simulink subsystem "est_observer"  (R2023a)
settings: Solver=VariableStepAuto  StartTime=0.0  StopTime=10.0  RelTol=1e-3
undefined symbols (not defined in the file or in its folder): ctrlP
libraries: simulink x1
settings Model: Creator=ahmad  LastModifiedBy=ahmad
settings ModelReferenceCC: UpdateModelReferenceTargets=IfOutOfDate
settings RTWCC: GPUComputeCapability=5.0
settings ConfigComp: CovBoundaryAbsTol=1.0e-5

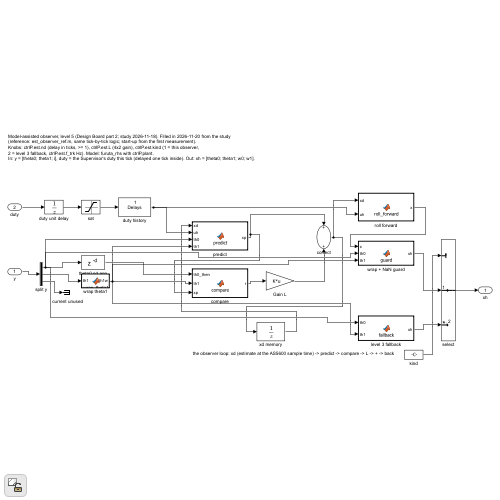
[thumbnail: Simulink's stored preview of the top-level diagram]
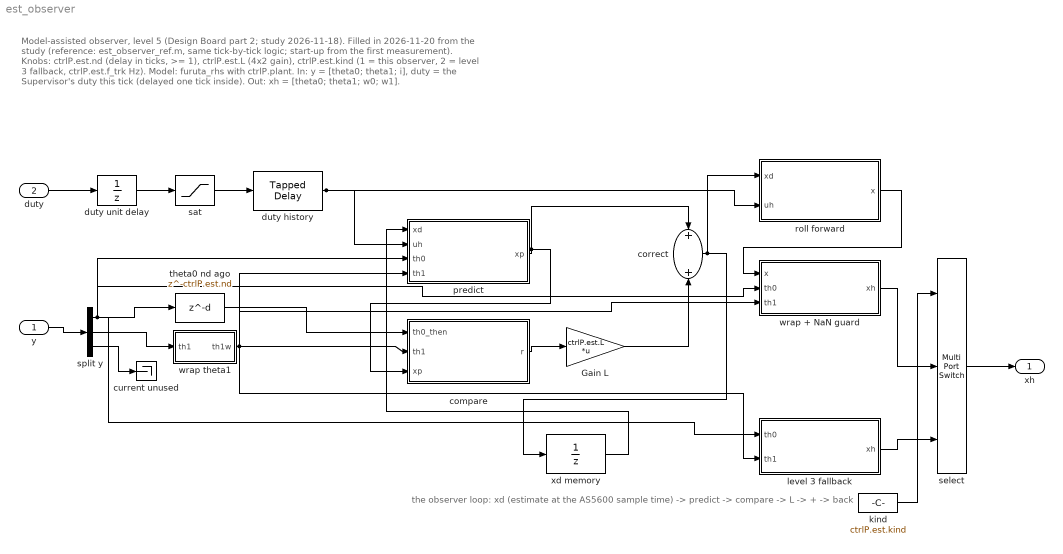
== system est_observer ==
  note: Model-assisted observer, level 5 (Design Board part 2; study 2026-11-18). Filled in 2026-11-20 from the study
      | (reference: est_observer_ref.m, same tick-by-tick logic; start-up from the first measurement).
      | Knobs: ctrlP.est.nd (delay in ticks, >= 1), ctrlP.est.L (4x2 gain), ctrlP.est.kind (1 = this observer,
      | 2 = level 3 fallback, ctrlP.est.f_trk Hz). Model: furuta_rhs with ctrlP.plant.
      | In: y = [theta0; theta1; i], duty = the Supervisor's duty this tick (delayed one tick inside). Out: xh = [theta0; theta1; w0; w1].
  note: the observer loop: xd (estimate at the AS5600 sample time) -> predict -> compare -> L -> + -> back
  y : Inport
  duty : Inport  Port=2
  Gain L : Gain  Gain=ctrlP.est.L  Multiplication=Matrix(K*u)
  compare : MATLAB Function  TreatAsAtomicUnit=on
  correct : Sum
  current unused : Terminator
  duty history : simulink/Discrete/Tapped Delay  vinit=0  samptime=ctrlP.Ts  NumDelays=ctrlP.est.nd  DelayOrder=Oldest  includeCurrent=on
  duty unit delay : UnitDelay  SampleTime=ctrlP.Ts
  kind : Constant  Value=ctrlP.est.kind
  level 3 fallback : MATLAB Function  TreatAsAtomicUnit=on
  predict : MATLAB Function  TreatAsAtomicUnit=on
  roll forward : MATLAB Function  TreatAsAtomicUnit=on
  sat : Saturate
  select : MultiPortSwitch  Inputs=2  SaturateOnIntegerOverflow=off  InputSameDT=off
  split y : Demux  Outputs=3
  theta0 nd ago : Delay  DelayLength=ctrlP.est.nd  InitialCondition=0  SampleTime=ctrlP.Ts
  wrap + NaN guard : MATLAB Function  TreatAsAtomicUnit=on
  wrap theta1 : MATLAB Function  TreatAsAtomicUnit=on
  xd memory : UnitDelay  InitialCondition=[0; pi; 0; 0]  SampleTime=ctrlP.Ts
  xh : Outport
  wires:
  y/1 -> split y/1
  split y/3 -> current unused/1
  split y/1 -> theta0 nd ago/1, wrap + NaN guard/2(th0), level 3 fallback/1(th0), predict/3(th0)
  split y/2 -> wrap theta1/1(th1)
  duty/1 -> duty unit delay/1
  duty unit delay/1 -> sat/1
  sat/1 -> duty history/1
  xd memory/1 -> predict/1(xd)
  duty history/1 -> predict/2(uh), roll forward/2(uh)
  theta0 nd ago/1 -> compare/1(th0_then)
  wrap theta1/1(th1w) -> compare/2(th1), wrap + NaN guard/3(th1), level 3 fallback/2(th1), predict/4(th1)
  predict/1(xp) -> compare/3(xp), correct/1
  compare/1(r) -> Gain L/1
  Gain L/1 -> correct/2
  correct/1 -> xd memory/1, roll forward/1(xd)
  roll forward/1(x) -> wrap + NaN guard/1(x)
  kind/1 -> select/1
  wrap + NaN guard/1(xh) -> select/2
  level 3 fallback/1(xh) -> select/3
  select/1 -> xh/1

== matlab function est_observer/predict ==
  data: xd input; xp output; uh input; th0 input; th1 input; ctrlP parameter
function xp = predict(xd, uh, th0, th1, ctrlP)
% Step the estimate at the AS5600 sample time one tick forward with the model.
% xd : estimate at the previous sample time (xd memory)
% uh : duty history [oldest ... newest] (nd+1 values); the OLDEST one acted during this step
% th0, th1 : the readings now; used once, to start from the first measurement (speeds 0)
% One RK4 step of furuta_rhs over ctrlP.Ts, in ctrlP.est.sub substeps (2 in the 2026-11-18 study).
persistent started
if isempty(started), started = false; end
if ~started
    started = true;
    xp = [th0; th1; 0; 0];
    return
end
p = ctrlP.plant; h = ctrlP.Ts/ctrlP.est.sub;
xp = xd;
xp(2) = mod(xp(2) + pi, 2*pi) - pi;           % keep the memory bounded when the pendulum spins
for q = 1:ctrlP.est.sub
    k1 = furuta_rhs(xp, uh(1), p); k2 = furuta_rhs(xp + h/2*k1, uh(1), p);
    k3 = furuta_rhs(xp + h/2*k2, uh(1), p); k4 = furuta_rhs(xp + h*k3, uh(1), p);
    xp = xp + h/6*(k1 + 2*k2 + 2*k3 + k4);
end

== matlab function est_observer/wrap theta1 ==
  data: th1 input; th1w output
function th1w = wrap_theta1(th1)
% theta1 wrapped to [-pi, pi), 0 = upright
th1w = mod(th1 + pi, 2*pi) - pi;

== matlab function est_observer/compare ==
  data: th0_then input; r output; th1 input; xp input; ctrlP parameter
function r = compare(th0_then, th1, xp, ctrlP)
% miss = measured - predicted, for both angles (2x1). The pendulum miss is wrapped to [-pi, pi).
% For the first nd ticks "theta0 nd ago" is still its initial 0, not a reading: its miss is ignored.
persistent n
if isempty(n), n = 0; end
n = n + 1;
r = [th0_then - xp(1); mod(th1 - xp(2) + pi, 2*pi) - pi];
if n <= ctrlP.est.nd, r(1) = 0; end

== matlab function est_observer/roll forward ==
  data: xd input; x output; uh input; ctrlP parameter
function x = roll_forward(xd, uh, ctrlP)
% Roll a COPY of xd forward to now through the newer duties uh(2:end) (nd ticks, ctrlP.est.sub RK4 substeps each).
p = ctrlP.plant; h = ctrlP.Ts/ctrlP.est.sub;
x = xd;
for j = 2:numel(uh)
    for q = 1:ctrlP.est.sub
        k1 = furuta_rhs(x, uh(j), p); k2 = furuta_rhs(x + h/2*k1, uh(j), p);
        k3 = furuta_rhs(x + h/2*k2, uh(j), p); k4 = furuta_rhs(x + h*k3, uh(j), p);
        x = x + h/6*(k1 + 2*k2 + 2*k3 + k4);
    end
end

== matlab function est_observer/wrap + NaN guard ==
  data: x input; xh output; th0 input; th1 input
function xh = guard(x, th0, th1)
% Wrap theta1 to [-pi, pi); if the estimate is not finite, fall back to the readings with speeds 0.
xh = x;
xh(2) = mod(xh(2) + pi, 2*pi) - pi;
if any(~isfinite(xh))
    xh = [th0; th1; 0; 0];
end

== matlab function est_observer/level 3 fallback ==
  data: th0 input; xh output; th1 input; ctrlP parameter
function xh = fallback(th0, th1, ctrlP)
% Level 3: alpha-beta tracking loop on both angles (critically damped, ctrlP.est.f_trk Hz), with
% theta1 pushed forward by the lag (nd ticks) using its speed. No model.
persistent th w
if isempty(th), th = [th0; th1]; w = [0; 0]; end
Ts = ctrlP.Ts;
lam = exp(-2*pi*ctrlP.est.f_trk*Ts); al = 1 - lam^2; be = (1 - lam)^2;
thp = th + Ts*w;
r = [th0; th1] - thp; r(2) = mod(r(2) + pi, 2*pi) - pi;
th = thp + al*r; th(2) = mod(th(2) + pi, 2*pi) - pi;
w = w + be/Ts*r;
xh = [th(1); mod(th(2) + w(2)*ctrlP.est.nd*Ts + pi, 2*pi) - pi; w];
